simulink model "BalancingBike"  (R2024b)
settings: Solver=FixedStepDiscrete  StartTime=0.0  StopTime=inf  FixedStep=0.005  RelTol=1e-3  EnableMultiTasking=on
undefined symbols (not defined in the file): dspblkCoreblockFVToolHelper, gcbh
libraries: mbedblockslib x10, simulink x8
settings Model: ExtModeTrigDuration=10  Creator=ACER  LastModifiedBy=QUANG
settings OptimizationCC: EnhancedBackFolding=on  PassReuseOutputArgsAs=Individual arguments  ZeroExternalMemoryAtStartup=off  ZeroInternalMemoryAtStartup=off  MaxStackSize=64  OptimizeBlockOrder=speed  DifferentSizesBufferReuse=on  OptimizationCustomize=off  EfficientTunableParamExpr=on
settings DebuggingCC: ParameterTunabilityLossMsg=error
settings HardwareCC: ProdBitPerPointer=32  ProdBitPerSizeT=32  ProdBitPerPtrDiffT=32  ProdLargestAtomicInteger=Long  ProdLargestAtomicFloat=Double  ProdWordSize=32  ProdLongLongMode=on  ProdHWDeviceType=ARM Compatible->ARM Cortex
settings SFSimCC: MATLABDynamicMemAlloc=off
settings RTWCC: Description=Embedded Coder  SystemTargetFile=ert.tlc  HardwareBoard=STM32 Nucleo F411RE  TemplateMakefile=ert_default_tmf  Toolchain=GNU Tools for ARM Embedded Processors  GPUComputeCapability=3.5
settings CodeAppCC: ForceParamTrailComments=on  IgnoreCustomStorageClasses=off  OperatorAnnotations=on  SimulinkDataObjDesc=on  SFDataObjDesc=on  InsertBlockDesc=on
settings ERTTargetCC: ExtModeTransport=3  ExtModeStaticAlloc=on  ExtModeStaticAllocSize=115200  ExtModeMexFile=ext_xcp  ExtModeIntrfLevel=Level2 - Open  InlinedParameterPlacement=Hierarchical  DynamicArrayContainerType=coder::array

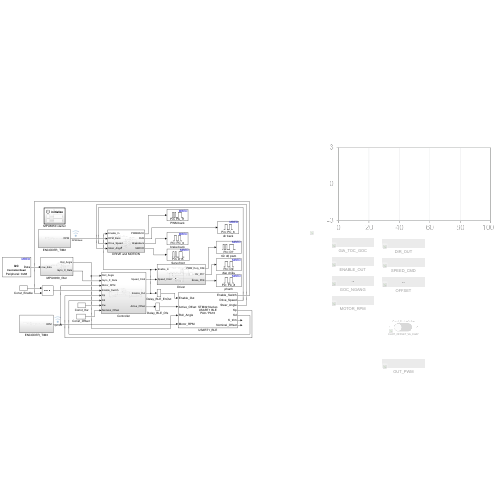
[thumbnail: Simulink's stored preview of the top-level diagram]
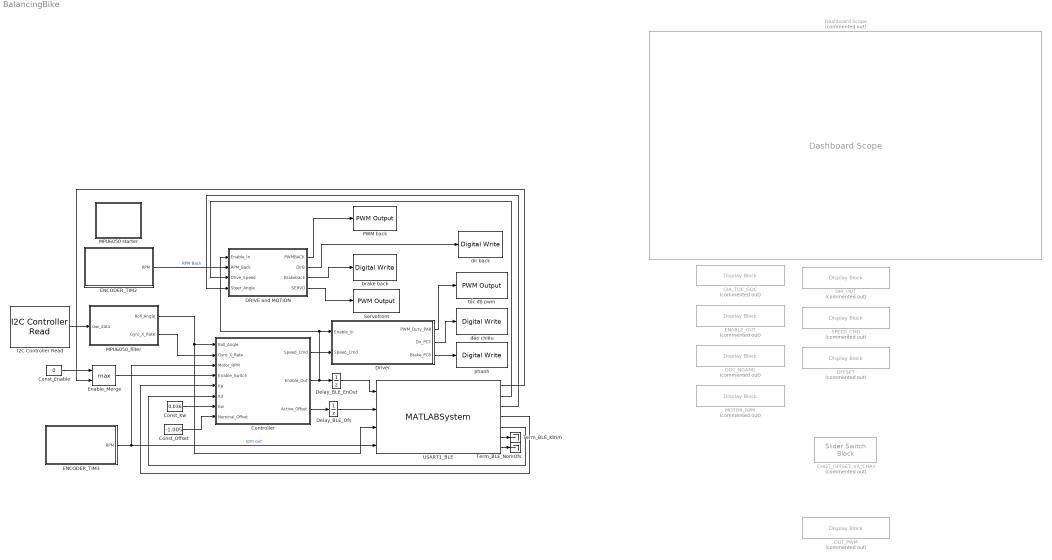
== system BalancingBike ==
  CHOT_OFFSET_VA_CHAY : SliderSwitchBlock  Commented=on
      settings: Values={{'Off', 'On'}, [0 1]}
  Const_Enable : Constant  Value=0  OutDataTypeStr=double
  Const_Kw : Constant  Value=0.036  OutDataTypeStr=double
  Const_Offset : Constant  Value=-1.005  OutDataTypeStr=double
  Controller : Subsystem
  DIR_OUT : DisplayBlock  Commented=on  LabelPosition=Hide  Transparency=1
  DRIVE and MOTION : Subsystem
  Dashboard Scope : DashboardScope  Commented=on
  Delay_BLE_EnOut : UnitDelay  InitialCondition=0.0  SampleTime=0.005  HasFrameUpgradeWarning=on
  Delay_BLE_Ofs : UnitDelay  InitialCondition=-1.005  SampleTime=0.005  HasFrameUpgradeWarning=on
  Driver : Subsystem
  ENABLE_OUT : DisplayBlock  Commented=on  LabelPosition=Hide  Transparency=1
  ENCODER_TIM2 : Subsystem
  "ENCODER_TIM3 " : Subsystem
  Enable_Merge : MinMax  Function=max  Inputs=2
  GIA_TOC_GOC : DisplayBlock  Commented=on  LabelPosition=Hide  Transparency=1
  GOC_NGANG : DisplayBlock  Commented=on  LabelPosition=Hide  Transparency=1
  I2C Controller Read : mbedblockslib/I2C Controller Read  I2CModule=0  Mode=Master  SlaveAddress=hex2dec('68')  SlaveByteOrder=BigEndian  Direction=Receiver  RegisterAddressMode=on  RegisterAddress=hex2dec('3B')  SlaveDataType=uint8  DataLength=14  NoAck=off  RepeatedStart=off  OutputStatus=off  SampleTime=0.005
      settings: LibrarySourceBlock=stmnucleorootlib/Common/I2C Controller Read
  MOTOR_RPM : DisplayBlock  Commented=on  LabelPosition=Hide  Transparency=1
  MPU6050 starter : Subsystem  TreatAsAtomicUnit=on
  MPU6050_filter : Subsystem
  OFFSET : DisplayBlock  Commented=on  LabelPosition=Hide  Transparency=1
  OUT_PWM : DisplayBlock  Commented=on  LabelPosition=Hide  Transparency=1
  PWM back : mbedblockslib/PWM Output  Pin=PA_11  EnableInputFrequency=off  InitialFrequency=20000  InitialDutyCycle=100  NotificationType=None
      settings: LibrarySourceBlock=stmnucleorootlib/Common/PWM Output
  SPEED_CMD : DisplayBlock  Commented=on  LabelPosition=Hide  Transparency=1
  Servofront : mbedblockslib/PWM Output  Pin=D15  EnableInputFrequency=off  InitialFrequency=50  InitialDutyCycle=100  NotificationType=None
      settings: LibrarySourceBlock=stmnucleorootlib/Common/PWM Output
  Term_BLE_Ktrim : Terminator
  Term_BLE_NomOfs : Terminator
  USART1_BLE : MATLABSystem  System=USART1Block_BLE  SampleTime=0.005
      mask Type: USART1Block_BLE
      mask Display:
      | disp(['STM32 Nucleo' char(10) 'USART1 BLE' char(10) 'PA9 / PA10']);
      | port_label('input',1,'Enable_Out');
      | port_label('input',2,'Active_Offset');
      | port_label('input',3,'Roll_Angle');
      | port_label('input',4,'Motor_RPM');
      | port_label('output',1,'Enable_Switch');
      | port_label('output',2,'Drive_Speed');
      | port_label('output',3,'Steer_Angle');
      | port_label('output',4,'Kp');
      | port_label('output',5,'Kd');
      | port_label('output',6,'K_trim');
      | port_label('output',7,'Nominal_Offset');
  brake back : mbedblockslib/Digital Write  Pin=PC_9  Direction=output
      settings: LibrarySourceBlock=stmnucleorootlib/Common/Digital Write
  dir back : mbedblockslib/Digital Write  Pin=PC_6  Direction=output
      settings: LibrarySourceBlock=stmnucleorootlib/Common/Digital Write
  phanh : mbedblockslib/Digital Write  Pin=PC_8  Direction=output
      settings: LibrarySourceBlock=stmnucleorootlib/Common/Digital Write
  tốc độ pwm : mbedblockslib/PWM Output  Pin=D7  EnableInputFrequency=off  InitialFrequency=20000  InitialDutyCycle=100  NotificationType=None
      settings: LibrarySourceBlock=stmnucleorootlib/Common/PWM Output
  đảo chiều : mbedblockslib/Digital Write  Pin=D9  Direction=output
      settings: LibrarySourceBlock=stmnucleorootlib/Common/Digital Write
  wires:
  Const_Offset/1 -> Controller/8(Nominal_Offset)
  Const_Enable/1 -> Enable_Merge/1
  I2C Controller Read/1 -> MPU6050_filter/1(raw_data)
  MPU6050_filter/2(Gyro_X_Rate) -> Controller/2(Gyro_X_Rate)
  Driver/1(PWM_Duty_PA8) -> tốc độ pwm/1
  USART1_BLE/2 -> DRIVE and MOTION/3(Drive_Speed)
  USART1_BLE/6 -> Term_BLE_Ktrim/1
  USART1_BLE/1 -> Enable_Merge/2
  USART1_BLE/4 -> Controller/5(Kp)
  USART1_BLE/5 -> Controller/6(Kd)
  USART1_BLE/3 -> DRIVE and MOTION/4(Steer_Angle)
  Enable_Merge/1 -> Controller/4(Enable_Switch)
  Const_Kw/1 -> Controller/7(Kw)
  ENCODER_TIM2/1("RPM ") -> DRIVE and MOTION/2(RPM_Back)  "RPM Back"
  Controller/1(Speed_Cmd) -> Driver/2(Speed_Cmd)
  Delay_BLE_Ofs/1 -> USART1_BLE/2
  Controller/2(Enable_Out) -> DRIVE and MOTION/1(Enable_In), Driver/1(Enable_In), Delay_BLE_EnOut/1
  Driver/3(Brake_PC8) -> phanh/1
  Controller/3(Active_Offset) -> Delay_BLE_Ofs/1
  DRIVE and MOTION/1(PWMBACK) -> PWM back/1
  DRIVE and MOTION/2(DirB) -> dir back/1
  DRIVE and MOTION/3(Brakeback) -> brake back/1
  DRIVE and MOTION/4(SERVO) -> Servofront/1
  Delay_BLE_EnOut/1 -> USART1_BLE/1
  Driver/2(Dir_PC7) -> đảo chiều/1
  USART1_BLE/7 -> Term_BLE_NomOfs/1
  "ENCODER_TIM3 "/1("RPM ") -> USART1_BLE/4, Controller/3(Motor_RPM)  "rpm out"
  MPU6050_filter/1(Roll_Angle) -> USART1_BLE/3, Controller/1(Roll_Angle)

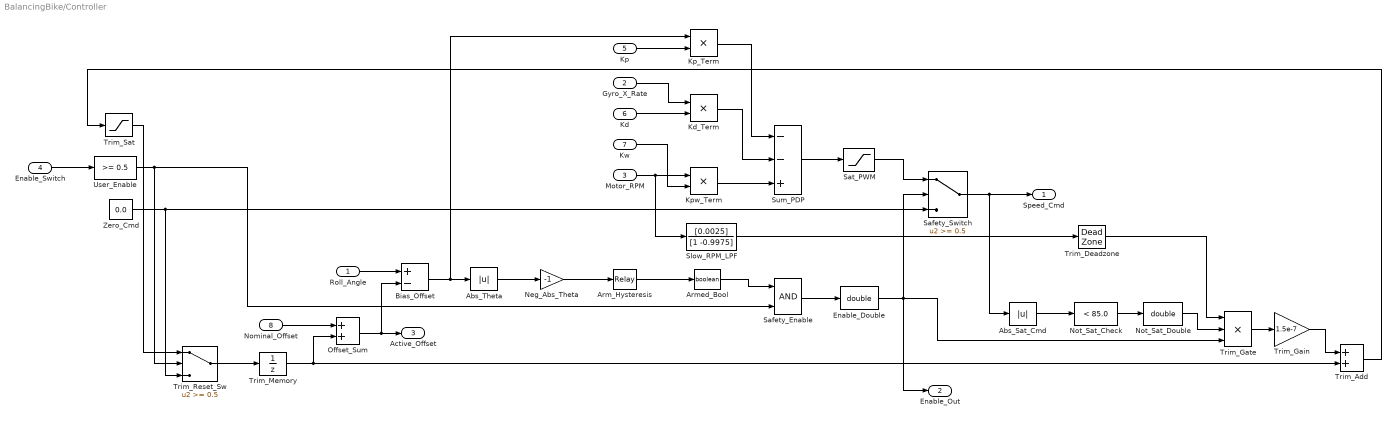
== system BalancingBike/Controller ==
  Roll_Angle : Inport
  Gyro_X_Rate : Inport  Port=2
  Motor_RPM : Inport  Port=3
  Enable_Switch : Inport  Port=4
  Kp : Inport  Port=5
  Kd : Inport  Port=6
  Kw : Inport  Port=7
  Nominal_Offset : Inport  Port=8
  Abs_Sat_Cmd : Abs  SaturateOnIntegerOverflow=off
  Abs_Theta : Abs  SaturateOnIntegerOverflow=off
  Arm_Hysteresis : Relay  OnSwitchValue=-2.0  OffSwitchValue=-12.0  ZeroCross=off
  Armed_Bool : DataTypeConversion  OutDataTypeStr=boolean
  Bias_Offset : Sum  Inputs=+-
  Enable_Double : DataTypeConversion  OutDataTypeStr=double  SaturateOnIntegerOverflow=off  RndMeth=Floor
  Kd_Term : Product
  Kp_Term : Product
  Kpw_Term : Product
  Neg_Abs_Theta : Gain  Gain=-1
  Not_Sat_Check : simulink/Logic and Bit Operations/Compare To Constant  relop=<  const=85.0  OutDataTypeStr=boolean
  Not_Sat_Double : DataTypeConversion  OutDataTypeStr=double  SaturateOnIntegerOverflow=off  RndMeth=Floor
  Offset_Sum : Sum
  Safety_Enable : Logic  AllPortsSameDT=off  OutDataTypeStr=boolean
  Safety_Switch : Switch  Threshold=0.5  SaturateOnIntegerOverflow=off  InputSameDT=off
  Sat_PWM : Saturate  UpperLimit=95.0  LowerLimit=-95.0
  Slow_RPM_LPF : DiscreteFilter  LoadFcn=dspblkCoreblockFVToolHelper(gcbh,'load');  Numerator=[0.0025]  Denominator=[1 -0.9975]  SampleTime=0.005
      settings: CopyFcn=dspblkCoreblockFVToolHelper(gcbh,'copy');  DeleteFcn=dspblkCoreblockFVToolHelper(gcbh,'close');  ModelCloseFcn=dspblkCoreblockFVToolHelper(gcbh,'close');  PreSaveFcn=dspblkCoreblockFVToolHelper(gcbh,'presave');  PostSaveFcn=dspblkCoreblockFVToolHelper(gcbh,'postsave');  CloseFcn=dspblkCoreblockFVToolHelper(gcbh,'close');
  Sum_PDP : Sum  Inputs=--+
  Trim_Add : Sum
  Trim_Deadzone : DeadZone  LowerValue=-30.0  UpperValue=30.0
  Trim_Gain : Gain  Gain=1.5e-7
  Trim_Gate : Product  Inputs=3
  Trim_Memory : UnitDelay  InitialCondition=0.0  SampleTime=-1  HasFrameUpgradeWarning=on
  Trim_Reset_Sw : Switch  Threshold=0.5  SaturateOnIntegerOverflow=off  InputSameDT=off
  Trim_Sat : Saturate  UpperLimit=1.5  LowerLimit=-1.5
  User_Enable : simulink/Logic and Bit Operations/Compare To Constant  relop=>=  const=0.5  OutDataTypeStr=boolean
  Zero_Cmd : Constant  Value=0.0  OutDataTypeStr=double
  Speed_Cmd : Outport
  Enable_Out : Outport  Port=2
  Active_Offset : Outport  Port=3
  wires:
  Enable_Double/1 -> Trim_Gate/3, Enable_Out/1, Safety_Switch/2
  Trim_Memory/1 -> Trim_Add/2, Offset_Sum/2
  Trim_Add/1 -> Trim_Sat/1
  Enable_Switch/1 -> User_Enable/1
  Trim_Reset_Sw/1 -> Trim_Memory/1
  Trim_Sat/1 -> Trim_Reset_Sw/1
  Roll_Angle/1 -> Bias_Offset/1
  Armed_Bool/1 -> Safety_Enable/1
  User_Enable/1 -> Trim_Reset_Sw/2, Safety_Enable/2
  Zero_Cmd/1 -> Safety_Switch/3, Trim_Reset_Sw/3
  Kd/1 -> Kd_Term/2
  Nominal_Offset/1 -> Offset_Sum/1
  Not_Sat_Double/1 -> Trim_Gate/2
  Safety_Enable/1 -> Enable_Double/1
  Offset_Sum/1 -> Bias_Offset/2, Active_Offset/1
  Bias_Offset/1 -> Kp_Term/1, Abs_Theta/1
  Kp/1 -> Kp_Term/2
  Abs_Theta/1 -> Neg_Abs_Theta/1
  Neg_Abs_Theta/1 -> Arm_Hysteresis/1
  Gyro_X_Rate/1 -> Kd_Term/1
  Kw/1 -> Kpw_Term/2
  Motor_RPM/1 -> Kpw_Term/1, Slow_RPM_LPF/1
  Arm_Hysteresis/1 -> Armed_Bool/1
  Kp_Term/1 -> Sum_PDP/1
  Kd_Term/1 -> Sum_PDP/2
  Kpw_Term/1 -> Sum_PDP/3
  Slow_RPM_LPF/1 -> Trim_Deadzone/1
  Sum_PDP/1 -> Sat_PWM/1
  Sat_PWM/1 -> Safety_Switch/1
  Safety_Switch/1 -> Speed_Cmd/1, Abs_Sat_Cmd/1
  Abs_Sat_Cmd/1 -> Not_Sat_Check/1
  Trim_Deadzone/1 -> Trim_Gate/1
  Not_Sat_Check/1 -> Not_Sat_Double/1
  Trim_Gate/1 -> Trim_Gain/1
  Trim_Gain/1 -> Trim_Add/1

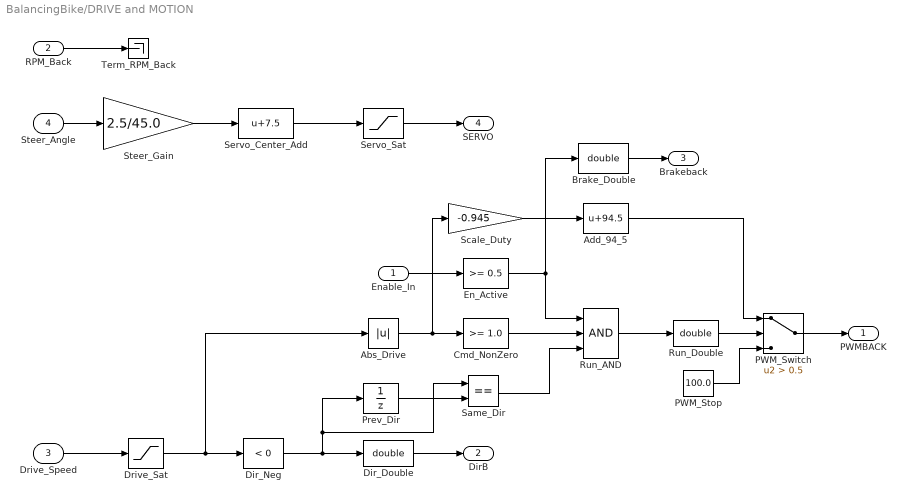
== system BalancingBike/DRIVE and MOTION ==
  Enable_In : Inport
  RPM_Back : Inport  Port=2
  Drive_Speed : Inport  Port=3
  Steer_Angle : Inport  Port=4
  Abs_Drive : Abs  SaturateOnIntegerOverflow=off
  Add_94_5 : Bias  Bias=94.5  SaturateOnIntegerOverflow=off
  Brake_Double : DataTypeConversion  OutDataTypeStr=double  SaturateOnIntegerOverflow=off  RndMeth=Floor
  Cmd_NonZero : simulink/Logic and Bit Operations/Compare To Constant  relop=>=  const=1.0  OutDataTypeStr=boolean
  Dir_Double : DataTypeConversion  OutDataTypeStr=double  SaturateOnIntegerOverflow=off  RndMeth=Floor
  Dir_Neg : simulink/Logic and Bit Operations/Compare To Constant  relop=<  const=0  OutDataTypeStr=boolean
  Drive_Sat : Saturate  UpperLimit=100.0  LowerLimit=-100.0
  En_Active : simulink/Logic and Bit Operations/Compare To Constant  relop=>=  const=0.5  OutDataTypeStr=boolean
  PWM_Stop : Constant  Value=100.0
  PWM_Switch : Switch  Criteria=u2 > Threshold  Threshold=0.5  SaturateOnIntegerOverflow=off  InputSameDT=off
  Prev_Dir : UnitDelay  SampleTime=-1  HasFrameUpgradeWarning=on
  Run_AND : Logic  Inputs=3  AllPortsSameDT=off  OutDataTypeStr=boolean
  Run_Double : DataTypeConversion  OutDataTypeStr=double  SaturateOnIntegerOverflow=off  RndMeth=Floor
  Same_Dir : RelationalOperator  Operator===  OutDataTypeStr=boolean  RndMeth=Simplest  InputSameDT=off
  Scale_Duty : Gain  Gain=-0.945
  Servo_Center_Add : Bias  Bias=7.5  SaturateOnIntegerOverflow=off
  Servo_Sat : Saturate  UpperLimit=10.0  LowerLimit=5.0
  Steer_Gain : Gain  Gain=2.5/45.0
  Term_RPM_Back : Terminator
  PWMBACK : Outport
  DirB : Outport  Port=2
  Brakeback : Outport  Port=3
  SERVO : Outport  Port=4
  wires:
  Enable_In/1 -> En_Active/1
  Drive_Speed/1 -> Drive_Sat/1
  RPM_Back/1 -> Term_RPM_Back/1
  Steer_Angle/1 -> Steer_Gain/1
  Servo_Sat/1 -> SERVO/1
  Steer_Gain/1 -> Servo_Center_Add/1
  Dir_Neg/1 -> Same_Dir/1, Prev_Dir/1, Dir_Double/1
  Drive_Sat/1 -> Abs_Drive/1, Dir_Neg/1
  Servo_Center_Add/1 -> Servo_Sat/1
  Abs_Drive/1 -> Scale_Duty/1, Cmd_NonZero/1
  PWM_Stop/1 -> PWM_Switch/3
  Run_Double/1 -> PWM_Switch/2
  Prev_Dir/1 -> Same_Dir/2
  Dir_Double/1 -> DirB/1
  Scale_Duty/1 -> Add_94_5/1
  En_Active/1 -> Brake_Double/1, Run_AND/1
  Cmd_NonZero/1 -> Run_AND/2
  Run_AND/1 -> Run_Double/1
  Same_Dir/1 -> Run_AND/3
  Brake_Double/1 -> Brakeback/1
  Add_94_5/1 -> PWM_Switch/1
  PWM_Switch/1 -> PWMBACK/1

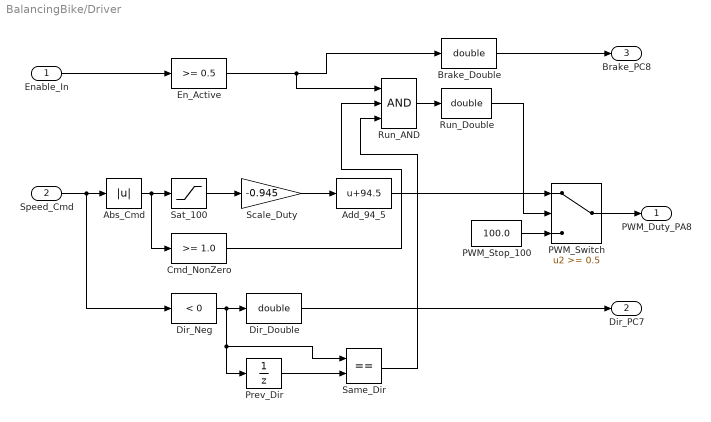
== system BalancingBike/Driver ==
  Enable_In : Inport
  Speed_Cmd : Inport  Port=2
  Abs_Cmd : Abs  SaturateOnIntegerOverflow=off
  Add_94_5 : Bias  Bias=94.5  SaturateOnIntegerOverflow=off
  Brake_Double : DataTypeConversion  OutDataTypeStr=double  SaturateOnIntegerOverflow=off  RndMeth=Floor
  Cmd_NonZero : simulink/Logic and Bit Operations/Compare To Constant  relop=>=  const=1.0  OutDataTypeStr=boolean
  Dir_Double : DataTypeConversion  OutDataTypeStr=double  SaturateOnIntegerOverflow=off  RndMeth=Floor
  Dir_Neg : simulink/Logic and Bit Operations/Compare To Zero  relop=<  OutDataTypeStr=boolean
  En_Active : simulink/Logic and Bit Operations/Compare To Constant  relop=>=  const=0.5  OutDataTypeStr=boolean
  PWM_Stop_100 : Constant  Value=100.0  OutDataTypeStr=double
  PWM_Switch : Switch  Threshold=0.5  SaturateOnIntegerOverflow=off  InputSameDT=off
  Prev_Dir : UnitDelay  InitialCondition=false  SampleTime=-1  HasFrameUpgradeWarning=on
  Run_AND : Logic  Inputs=3  AllPortsSameDT=off  OutDataTypeStr=boolean
  Run_Double : DataTypeConversion  OutDataTypeStr=double  SaturateOnIntegerOverflow=off  RndMeth=Floor
  Same_Dir : RelationalOperator  Operator===  OutDataTypeStr=boolean  RndMeth=Simplest  InputSameDT=off
  Sat_100 : Saturate  UpperLimit=100.0  LowerLimit=0.0
  Scale_Duty : Gain  Gain=-0.945
  PWM_Duty_PA8 : Outport
  Dir_PC7 : Outport  Port=2
  Brake_PC8 : Outport  Port=3
  wires:
  Speed_Cmd/1 -> Abs_Cmd/1, Dir_Neg/1
  Abs_Cmd/1 -> Sat_100/1, Cmd_NonZero/1
  Sat_100/1 -> Scale_Duty/1
  Scale_Duty/1 -> Add_94_5/1
  Dir_Neg/1 -> Prev_Dir/1, Same_Dir/1, Dir_Double/1
  Prev_Dir/1 -> Same_Dir/2
  Enable_In/1 -> En_Active/1
  En_Active/1 -> Run_AND/1, Brake_Double/1
  Cmd_NonZero/1 -> Run_AND/2
  Same_Dir/1 -> Run_AND/3
  Run_AND/1 -> Run_Double/1
  Add_94_5/1 -> PWM_Switch/1
  Run_Double/1 -> PWM_Switch/2
  PWM_Stop_100/1 -> PWM_Switch/3
  PWM_Switch/1 -> PWM_Duty_PA8/1
  Dir_Double/1 -> Dir_PC7/1
  Brake_Double/1 -> Brake_PC8/1

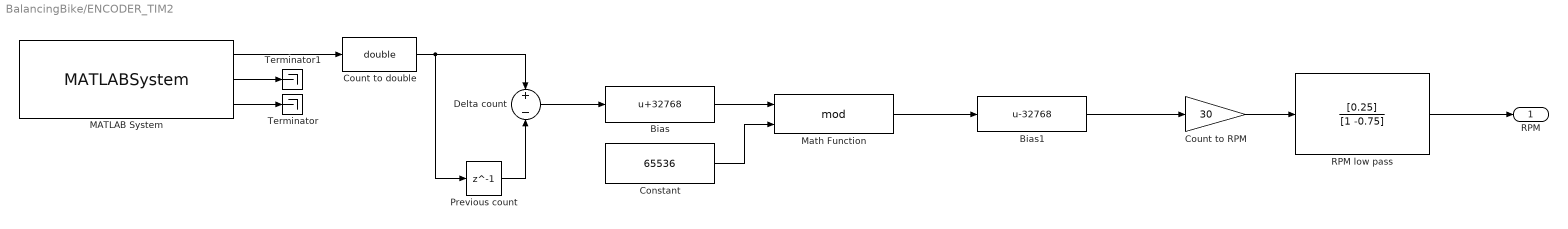
== system BalancingBike/ENCODER_TIM2 ==
  Bias : Bias  Bias=32768  SaturateOnIntegerOverflow=off
  Bias1 : Bias  Bias=-32768  SaturateOnIntegerOverflow=off
  Constant : Constant  Value=65536
  Count to RPM : Gain  Gain=30
  Count to double : DataTypeConversion  OutDataTypeStr=double  SaturateOnIntegerOverflow=off  RndMeth=Floor
  Delta count : Sum  Inputs=+-
  MATLAB System : MATLABSystem  System=EncoderBlock_TIM2  SampleTime=0.005
      mask Type: EncoderBlock_TIM2
      mask Display:
      | disp(['STM32 Nucleo' char(10) 'Encoder TIM2' char(10) '(PA15 / PB3)']);
      | port_label('output',1,'EncoderCount');
      | port_label('output',2,'IndexCount');
      | port_label('output',3,'ValidIndex');
  Math Function : Math  Operator=mod
  Previous count : Delay  DelayLength=1  InitialCondition=0  SampleTime=0.005
  RPM low pass : DiscreteFilter  LoadFcn=dspblkCoreblockFVToolHelper(gcbh,'load');  Numerator=[0.25]  Denominator=[1 -0.75]
      settings: CopyFcn=dspblkCoreblockFVToolHelper(gcbh,'copy');  DeleteFcn=dspblkCoreblockFVToolHelper(gcbh,'close');  ModelCloseFcn=dspblkCoreblockFVToolHelper(gcbh,'close');  PreSaveFcn=dspblkCoreblockFVToolHelper(gcbh,'presave');  PostSaveFcn=dspblkCoreblockFVToolHelper(gcbh,'postsave');  CloseFcn=dspblkCoreblockFVToolHelper(gcbh,'close');
  Terminator : Terminator
  Terminator1 : Terminator
  "RPM " : Outport
  wires:
  Previous count/1 -> Delta count/2
  Count to double/1 -> Delta count/1, Previous count/1
  MATLAB System/1 -> Count to double/1
  Count to RPM/1 -> RPM low pass/1
  RPM low pass/1 -> "RPM "/1
  Delta count/1 -> Bias/1
  Bias/1 -> Math Function/1
  Constant/1 -> Math Function/2
  Math Function/1 -> Bias1/1
  Bias1/1 -> Count to RPM/1
  MATLAB System/3 -> Terminator/1
  MATLAB System/2 -> Terminator1/1

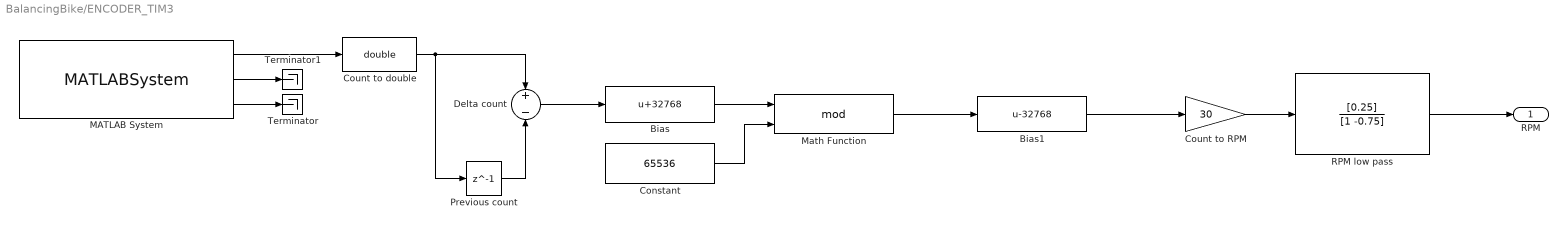
== system BalancingBike/ENCODER_TIM3  ==
  Bias : Bias  Bias=32768  SaturateOnIntegerOverflow=off
  Bias1 : Bias  Bias=-32768  SaturateOnIntegerOverflow=off
  Constant : Constant  Value=65536
  Count to RPM : Gain  Gain=30
  Count to double : DataTypeConversion  OutDataTypeStr=double  SaturateOnIntegerOverflow=off  RndMeth=Floor
  Delta count : Sum  Inputs=+-
  MATLAB System : MATLABSystem  System=EncoderBlock_TIM3  SampleTime=0.005
      mask Type: EncoderBlock_TIM3
      mask Display:
      | disp(['STM32 Nucleo' char(10) 'Encoder TIM3' char(10) '(PA6 / PA7)']);
      | port_label('output',1,'EncoderCount');
      | port_label('output',2,'IndexCount');
      | port_label('output',3,'ValidIndex');
  Math Function : Math  Operator=mod
  Previous count : Delay  DelayLength=1  InitialCondition=0  SampleTime=0.005
  RPM low pass : DiscreteFilter  LoadFcn=dspblkCoreblockFVToolHelper(gcbh,'load');  Numerator=[0.25]  Denominator=[1 -0.75]
      settings: CopyFcn=dspblkCoreblockFVToolHelper(gcbh,'copy');  DeleteFcn=dspblkCoreblockFVToolHelper(gcbh,'close');  ModelCloseFcn=dspblkCoreblockFVToolHelper(gcbh,'close');  PreSaveFcn=dspblkCoreblockFVToolHelper(gcbh,'presave');  PostSaveFcn=dspblkCoreblockFVToolHelper(gcbh,'postsave');  CloseFcn=dspblkCoreblockFVToolHelper(gcbh,'close');
  Terminator : Terminator
  Terminator1 : Terminator
  "RPM " : Outport
  wires:
  Previous count/1 -> Delta count/2
  Count to double/1 -> Delta count/1, Previous count/1
  MATLAB System/1 -> Count to double/1
  Count to RPM/1 -> RPM low pass/1
  RPM low pass/1 -> "RPM "/1
  Delta count/1 -> Bias/1
  Bias/1 -> Math Function/1
  Constant/1 -> Math Function/2
  Math Function/1 -> Bias1/1
  Bias1/1 -> Count to RPM/1
  MATLAB System/3 -> Terminator/1
  MATLAB System/2 -> Terminator1/1

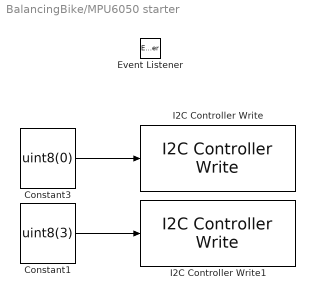
== system BalancingBike/MPU6050 starter ==
  Constant1 : Constant  Value=uint8(3)
  Constant3 : Constant  Value=uint8(0)
  Event Listener : EventListener  DisableCoverage=on  EventName=reset
  I2C Controller Write : mbedblockslib/I2C Controller Write  I2CModule=0  Mode=Master  SlaveAddress=hex2dec('68')  SlaveByteOrder=BigEndian  Direction=Transmitter  RegisterAddressMode=on  RegisterAddress=hex2dec('6B')  SlaveDataType=uint8  DataLength=2  NoAck=off  RepeatedStart=off  OutputStatus=on
      settings: LibrarySourceBlock=stmnucleorootlib/Common/I2C Controller Write
  I2C Controller Write1 : mbedblockslib/I2C Controller Write  I2CModule=0  Mode=Master  SlaveAddress=hex2dec('68')  SlaveByteOrder=BigEndian  Direction=Transmitter  RegisterAddressMode=on  RegisterAddress=hex2dec('1A')  SlaveDataType=uint8  DataLength=2  NoAck=off  RepeatedStart=off  OutputStatus=on
      settings: LibrarySourceBlock=stmnucleorootlib/Common/I2C Controller Write
  wires:
  Constant3/1 -> I2C Controller Write/1
  Constant1/1 -> I2C Controller Write1/1

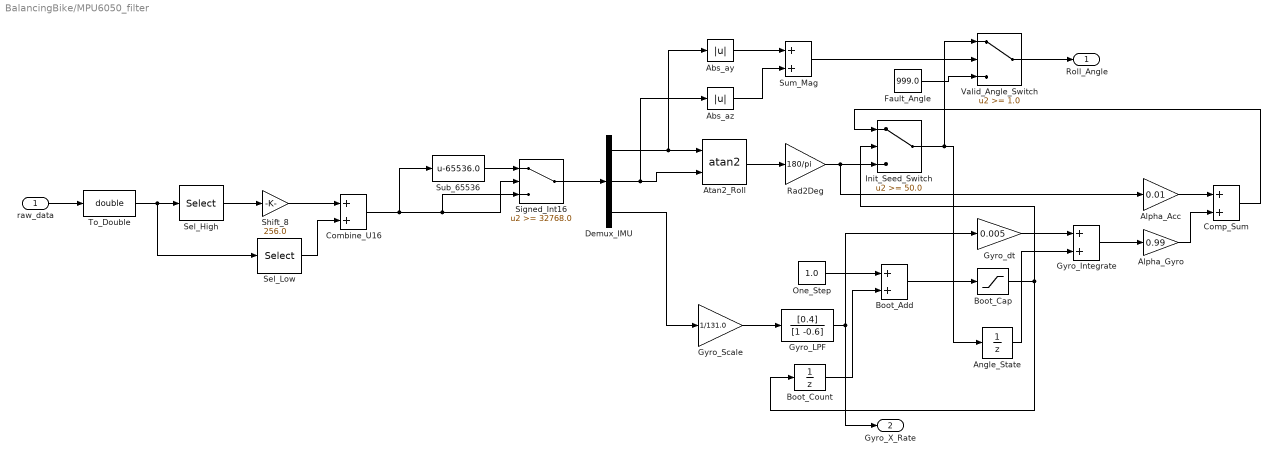
== system BalancingBike/MPU6050_filter ==
  raw_data : Inport
  Abs_ay : Abs  SaturateOnIntegerOverflow=off
  Abs_az : Abs  SaturateOnIntegerOverflow=off
  Alpha_Acc : Gain  Gain=0.01
  Alpha_Gyro : Gain  Gain=0.99
  Angle_State : UnitDelay  InitialCondition=1.35  SampleTime=-1  HasFrameUpgradeWarning=on
  Atan2_Roll : Trigonometry  Operator=atan2
  Boot_Add : Sum
  Boot_Cap : Saturate  UpperLimit=1000.0  LowerLimit=0.0
  Boot_Count : UnitDelay  InitialCondition=0.0  SampleTime=-1  HasFrameUpgradeWarning=on
  Combine_U16 : Sum
  Comp_Sum : Sum
  Demux_IMU : Demux  Outputs=3
  Fault_Angle : Constant  Value=999.0  OutDataTypeStr=double
  Gyro_Integrate : Sum
  Gyro_LPF : DiscreteFilter  Numerator=[0.4]  Denominator=[1 -0.6]  SampleTime=0.005
  Gyro_Scale : Gain  Gain=1/131.0
  Gyro_dt : Gain  Gain=0.005
  Init_Seed_Switch : Switch  Threshold=50.0  SaturateOnIntegerOverflow=off  InputSameDT=off
  One_Step : Constant  Value=1.0  OutDataTypeStr=double
  Rad2Deg : Gain  Gain=180/pi
  Sel_High : Selector  InputPortWidth=14  IndexOptions=Index vector (dialog)  Indices=[3 5 9]  OutputSizes=1
  Sel_Low : Selector  InputPortWidth=14  IndexOptions=Index vector (dialog)  Indices=[4 6 10]  OutputSizes=1
  Shift_8 : Gain  Gain=256.0
  Signed_Int16 : Switch  Threshold=32768.0  SaturateOnIntegerOverflow=off  InputSameDT=off
  Sub_65536 : Bias  Bias=-65536.0  SaturateOnIntegerOverflow=off
  Sum_Mag : Sum
  To_Double : DataTypeConversion  OutDataTypeStr=double  SaturateOnIntegerOverflow=off  RndMeth=Floor
  Valid_Angle_Switch : Switch  Threshold=1.0  SaturateOnIntegerOverflow=off  InputSameDT=off
  Roll_Angle : Outport
  Gyro_X_Rate : Outport  Port=2
  wires:
  Alpha_Gyro/1 -> Comp_Sum/2
  Demux_IMU/2 -> Atan2_Roll/2, Abs_az/1
  Combine_U16/1 -> Signed_Int16/2, Signed_Int16/3, Sub_65536/1
  Comp_Sum/1 -> Init_Seed_Switch/1
  Boot_Count/1 -> Boot_Add/2
  raw_data/1 -> To_Double/1
  Init_Seed_Switch/1 -> Angle_State/1, Valid_Angle_Switch/1
  Gyro_Scale/1 -> Gyro_LPF/1
  Sel_High/1 -> Shift_8/1
  To_Double/1 -> Sel_Low/1, Sel_High/1
  Sel_Low/1 -> Combine_U16/2
  Signed_Int16/1 -> Demux_IMU/1
  Shift_8/1 -> Combine_U16/1
  Sub_65536/1 -> Signed_Int16/1
  Gyro_Integrate/1 -> Alpha_Gyro/1
  Angle_State/1 -> Gyro_Integrate/2
  Demux_IMU/1 -> Atan2_Roll/1, Abs_ay/1
  Boot_Cap/1 -> Boot_Count/1, Init_Seed_Switch/2
  Demux_IMU/3 -> Gyro_Scale/1
  Fault_Angle/1 -> Valid_Angle_Switch/3
  Abs_ay/1 -> Sum_Mag/1
  Boot_Add/1 -> Boot_Cap/1
  Abs_az/1 -> Sum_Mag/2
  Gyro_LPF/1 -> Gyro_dt/1, Gyro_X_Rate/1
  Atan2_Roll/1 -> Rad2Deg/1
  Valid_Angle_Switch/1 -> Roll_Angle/1
  Sum_Mag/1 -> Valid_Angle_Switch/2
  Rad2Deg/1 -> Alpha_Acc/1, Init_Seed_Switch/3
  One_Step/1 -> Boot_Add/1
  Gyro_dt/1 -> Gyro_Integrate/1
  Alpha_Acc/1 -> Comp_Sum/1
